simulink model "untitled"  (R2025b)
settings: Solver=VariableStepAuto  StartTime=0.0  StopTime=26  RelTol=1e-3
libraries: neural x35
(part 2 of 2)

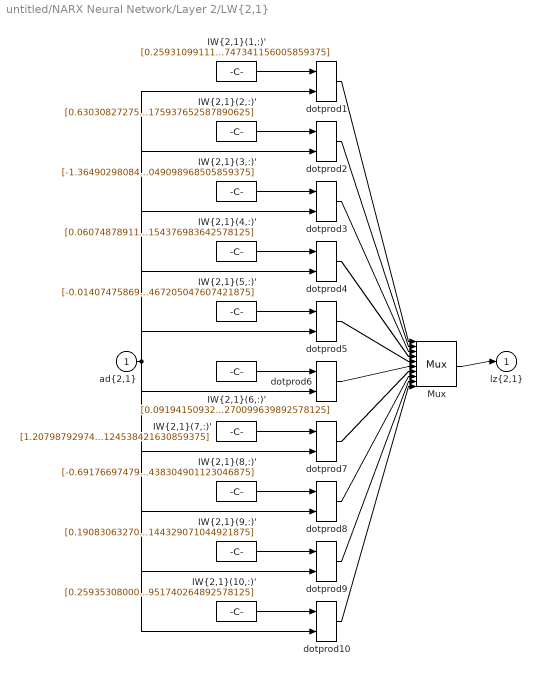
== system untitled/NARX Neural Network/Layer 2/LW{2,1} ==
  "ad{2,1}" : Inport  PortDimensions=10  SampleTime=1
      mask Display: e = 0.06;c1 = [120 230 180]/255;c2 = ([120 230 180]+0)/(256+128);c3 = ([120 230 180]+128)/(256+128);patch([0 1 1 0],[0 0 1 1],c1);patch([0 1 1 1-e 1-e 0+e],[0 0 1 1-e 0+e 0+e],c2);patch([0 0 1 1-e 0+e 0+e],[0 1 1 1-e 1-e 0+e],c3);plot([0 1 1 0 0],[0 0 1 1 0]);
  "IW{2,1}(1,:)'" : Constant  Value=[0.2593109911101532105703881825320422649383544921875;0.043027177460193015423595142010526615194976329803466796875;-0.031630578930780896274033153758864500559866428375244140625;-0.8946206870678163891597023393842391669750213623046875;-1.376635707680159637078531886800192296504974365234375;0.0101372112858142127134186694092932157218456268310546875;-0.036902676601514618204280537838712916709482669830322265625;0.07042545743955726245122406226073508150875568389892578125;0.126162243134557316981414487599977292120456695556640625;-0.6207380455155016019119784687063656747341156005859375]
      mask Display: e = 0.06;c1 = [120 150 230]/255;c2 = ([120 150 230]+0)/383;c3 = ([120 150 230]+128)/383;patch([0 1 1 0],[0 0 1 1],c1);patch([0 1 1 1-e 1-e 0+e],[0 0 1 1-e 0+e 0+e],c2);patch([0 0 1 1-e 0+e 0+e],[0 1 1 1-e 1-e 0+e],c3);plot([0 1 1 0 0],[0 0 1 1 0]);disp('weights');
  "IW{2,1}(10,:)'" : Constant  Value=[0.259353080009003644779141950493794865906238555908203125;0.0344788966224069126642604032895178534090518951416015625;-1.639734198097074990840837926953099668025970458984375;0.037171314064603451499113617728653480298817157745361328125;-0.044091665192930361294454399967435165308415889739990234375;0.113806681736434545104685867045191116631031036376953125;-0.0404618156560806740973390560611733235418796539306640625;0.0762493477749900117057535453568561933934688568115234375;-0.277877005672673871305988768654060550034046173095703125;0.047364494032463178019298766230349428951740264892578125]
      mask Display: e = 0.06;c1 = [120 150 230]/255;c2 = ([120 150 230]+0)/383;c3 = ([120 150 230]+128)/383;patch([0 1 1 0],[0 0 1 1],c1);patch([0 1 1 1-e 1-e 0+e],[0 0 1 1-e 0+e 0+e],c2);patch([0 0 1 1-e 0+e 0+e],[0 1 1 1-e 1-e 0+e],c3);plot([0 1 1 0 0],[0 0 1 1 0]);disp('weights');
  "IW{2,1}(2,:)'" : Constant  Value=[0.63030827275463219283579974216991104185581207275390625;0.95420909453976487935022987585398368537425994873046875;-0.0170684212993636071076242188837568392045795917510986328125;0.10423405085466287689488495971090742386877536773681640625;0.0933351443445988027125537200845428742468357086181640625;0.05706595557659464856836706303511164151132106781005859375;-0.0036970778483764979611969625494793945108540356159210205078125;0.0226284225386658120748872846661470248363912105560302734375;-0.169997488913500027774006184699828736484050750732421875;0.4467008606033611162189345122897066175937652587890625]
      mask Display: e = 0.06;c1 = [120 150 230]/255;c2 = ([120 150 230]+0)/383;c3 = ([120 150 230]+128)/383;patch([0 1 1 0],[0 0 1 1],c1);patch([0 1 1 1-e 1-e 0+e],[0 0 1 1-e 0+e 0+e],c2);patch([0 0 1 1-e 0+e 0+e],[0 1 1 1-e 1-e 0+e],c3);plot([0 1 1 0 0],[0 0 1 1 0]);disp('weights');
  "IW{2,1}(3,:)'" : Constant  Value=[-1.3649029808437316280134155022096820175647735595703125;-0.0099506250485993270882278949329702300019562244415283203125;0.004944580631372802632939045253124277223832905292510986328125;0.52636799453096261292017743471660651266574859619140625;0.0107608841966076625162873625640713726170361042022705078125;3.2396981083788300992409858736209571361541748046875;0.0175827063636769566346007565016407170332968235015869140625;-0.00844932741786058767730072105450744857080280780792236328125;-0.0488448562737805735967100417838082648813724517822265625;0.6284819327693680346413884763023816049098968505859375]
      mask Display: e = 0.06;c1 = [120 150 230]/255;c2 = ([120 150 230]+0)/383;c3 = ([120 150 230]+128)/383;patch([0 1 1 0],[0 0 1 1],c1);patch([0 1 1 1-e 1-e 0+e],[0 0 1 1-e 0+e 0+e],c2);patch([0 0 1 1-e 0+e 0+e],[0 1 1 1-e 1-e 0+e],c3);plot([0 1 1 0 0],[0 0 1 1 0]);disp('weights');
  "IW{2,1}(4,:)'" : Constant  Value=[0.060748789116446537394988780533822136931121349334716796875;-0.00794143061588940997463925697275044512934982776641845703125;-0.0246556586678514065569256530352504341863095760345458984375;-0.036168325016118781090046496728973579593002796173095703125;0.017769845931746054701338977110935957171022891998291015625;-0.00682202459217154215387335369769061799161136150360107421875;0.00478693571736033170183066687286554952152073383331298828125;1.828233176941406856741423325729556381702423095703125;-0.336457903351097209476705529596074484288692474365234375;-0.444354288008560083245157557030324824154376983642578125]
      mask Display: e = 0.06;c1 = [120 150 230]/255;c2 = ([120 150 230]+0)/383;c3 = ([120 150 230]+128)/383;patch([0 1 1 0],[0 0 1 1],c1);patch([0 1 1 1-e 1-e 0+e],[0 0 1 1-e 0+e 0+e],c2);patch([0 0 1 1-e 0+e 0+e],[0 1 1 1-e 1-e 0+e],c3);plot([0 1 1 0 0],[0 0 1 1 0]);disp('weights');
  "IW{2,1}(5,:)'" : Constant  Value=[-0.01407475869495870314518359833755312138237059116363525390625;-0.0813608715144924499185208333074115216732025146484375;0.1181201219432181648283375352548318915069103240966796875;0.76491096816797898849671355492318980395793914794921875;0.11204011842603171789090055199267226271331310272216796875;-0.385610136227055699809085353990667499601840972900390625;0.0940923757188020515318527259296388365328311920166015625;-0.152898200506478121329934083405532874166965484619140625;-0.0241401187729273873638913272543504717759788036346435546875;-1.02487649672637370912298138136975467205047607421875]
      mask Display: e = 0.06;c1 = [120 150 230]/255;c2 = ([120 150 230]+0)/383;c3 = ([120 150 230]+128)/383;patch([0 1 1 0],[0 0 1 1],c1);patch([0 1 1 1-e 1-e 0+e],[0 0 1 1-e 0+e 0+e],c2);patch([0 0 1 1-e 0+e 0+e],[0 1 1 1-e 1-e 0+e],c3);plot([0 1 1 0 0],[0 0 1 1 0]);disp('weights');
  "IW{2,1}(6,:)'" : Constant  Value=[0.09194150932908216888872487970729707740247249603271484375;0.00893170196256900909836939916885967249982059001922607421875;-0.00270216338763807316369902622454901575110852718353271484375;0.4384877115912220180149461157270707190036773681640625;-0.010539276489478908993557837447951897047460079193115234375;0.1074971903280156071414097596061765216290950775146484375;-0.0139268622037817708936291438703847234137356281280517578125;0.014467383049023820051903754801969625987112522125244140625;0.033730896861891353222251410670651239342987537384033203125;-0.47233994547981617007081922565703280270099639892578125]
      mask Display: e = 0.06;c1 = [120 150 230]/255;c2 = ([120 150 230]+0)/383;c3 = ([120 150 230]+128)/383;patch([0 1 1 0],[0 0 1 1],c1);patch([0 1 1 1-e 1-e 0+e],[0 0 1 1-e 0+e 0+e],c2);patch([0 0 1 1-e 0+e 0+e],[0 1 1 1-e 1-e 0+e],c3);plot([0 1 1 0 0],[0 0 1 1 0]);disp('weights');
  "IW{2,1}(7,:)'" : Constant  Value=[1.2079879297442683849794775596819818019866943359375;-0.96997720146081534142723512559314258396625518798828125;1.341993650625849188173788206768222153186798095703125;2.48313839798580904272284897160716354846954345703125;1.236241853293317038975374089204706251621246337890625;-2.98728747420875695439690389321185648441314697265625;0.99144276990696145190895549603737890720367431640625;-1.8470882435209095007166979485191404819488525390625;-0.39711441564978733342883288059965707361698150634765625;-1.9294405292739680302105398368439637124538421630859375]
      mask Display: e = 0.06;c1 = [120 150 230]/255;c2 = ([120 150 230]+0)/383;c3 = ([120 150 230]+128)/383;patch([0 1 1 0],[0 0 1 1],c1);patch([0 1 1 1-e 1-e 0+e],[0 0 1 1-e 0+e 0+e],c2);patch([0 0 1 1-e 0+e 0+e],[0 1 1 1-e 1-e 0+e],c3);plot([0 1 1 0 0],[0 0 1 1 0]);disp('weights');
  "IW{2,1}(8,:)'" : Constant  Value=[-0.6917669747991321838043177194776944816112518310546875;0.02005886442724380547275586650357581675052642822265625;0.2344520490258656664206426967211882583796977996826171875;0.16810169695141408130467652881634421646595001220703125;-0.0161572705531280273738570230079858447425067424774169921875;-0.1757694695147239138943717762231244705617427825927734375;-0.021758463862406492161927218376149539835751056671142578125;0.046202714262242240705891305196928442455828189849853515625;0.92224582634424034921494239824824035167694091796875;-0.57227723426191967615039857264491729438304901123046875]
      mask Display: e = 0.06;c1 = [120 150 230]/255;c2 = ([120 150 230]+0)/383;c3 = ([120 150 230]+128)/383;patch([0 1 1 0],[0 0 1 1],c1);patch([0 1 1 1-e 1-e 0+e],[0 0 1 1-e 0+e 0+e],c2);patch([0 0 1 1-e 0+e 0+e],[0 1 1 1-e 1-e 0+e],c3);plot([0 1 1 0 0],[0 0 1 1 0]);disp('weights');
  "IW{2,1}(9,:)'" : Constant  Value=[0.1908306327012936065568027288463781587779521942138671875;-0.0182508750380459862372450885459329583682119846343994140625;0.006372142546187395568957345659555357997305691242218017578125;-0.071890224988197803934752982968348078429698944091796875;0.044783945745097551716096262452992959879338741302490234375;0.026064510211621379209834259427225333638489246368408203125;-0.94180942639733522536715781825478188693523406982421875;-0.02284578978884177491437412754748947918415069580078125;-0.201690086770057452891791172078228555619716644287109375;0.63128763532050136131346107504214160144329071044921875]
      mask Display: e = 0.06;c1 = [120 150 230]/255;c2 = ([120 150 230]+0)/383;c3 = ([120 150 230]+128)/383;patch([0 1 1 0],[0 0 1 1],c1);patch([0 1 1 1-e 1-e 0+e],[0 0 1 1-e 0+e 0+e],c2);patch([0 0 1 1-e 0+e 0+e],[0 1 1 1-e 1-e 0+e],c3);plot([0 1 1 0 0],[0 0 1 1 0]);disp('weights');
  Mux : Mux  Inputs=10
      mask Display: e = 0.06;c1 = [120 150 230]/255;c2 = ([120 150 230]+0)/383;c3 = ([120 150 230]+128)/383;patch([0 1 1 0],[0 0 1 1],c1);patch([0 1 1 1-e 1-e 0+e],[0 0 1 1-e 0+e 0+e],c2);patch([0 0 1 1-e 0+e 0+e],[0 1 1 1-e 1-e 0+e],c3);plot([0 1 1 0 0],[0 0 1 1 0]);disp('Mux');
  dotprod{1..10} (10 alike) : neural/Weight Functions/dotprod
  "lz{2,1}" : Outport
      mask Display: e = 0.06;c1 = [120 230 180]/255;c2 = ([120 230 180]+0)/(256+128);c3 = ([120 230 180]+128)/(256+128);patch([0 1 1 0],[0 0 1 1],c1);patch([0 1 1 1-e 1-e 0+e],[0 0 1 1-e 0+e 0+e],c2);patch([0 0 1 1-e 0+e 0+e],[0 1 1 1-e 1-e 0+e],c3);plot([0 1 1 0 0],[0 0 1 1 0]);
  wires:
  "IW{2,1}(1,:)'"/1 -> dotprod1/1
  "ad{2,1}"/1 -> dotprod1/2, dotprod2/2, dotprod3/2, dotprod4/2, dotprod5/2, dotprod6/2, dotprod7/2, dotprod8/2, dotprod9/2, dotprod10/2
  dotprod1/1 -> Mux/1
  "IW{2,1}(2,:)'"/1 -> dotprod2/1
  dotprod2/1 -> Mux/2
  "IW{2,1}(3,:)'"/1 -> dotprod3/1
  dotprod3/1 -> Mux/3
  "IW{2,1}(4,:)'"/1 -> dotprod4/1
  dotprod4/1 -> Mux/4
  "IW{2,1}(5,:)'"/1 -> dotprod5/1
  dotprod5/1 -> Mux/5
  "IW{2,1}(6,:)'"/1 -> dotprod6/1
  dotprod6/1 -> Mux/6
  "IW{2,1}(7,:)'"/1 -> dotprod7/1
  dotprod7/1 -> Mux/7
  "IW{2,1}(8,:)'"/1 -> dotprod8/1
  dotprod8/1 -> Mux/8
  "IW{2,1}(9,:)'"/1 -> dotprod9/1
  dotprod9/1 -> Mux/9
  "IW{2,1}(10,:)'"/1 -> dotprod10/1
  dotprod10/1 -> Mux/10
  Mux/1 -> "lz{2,1}"/1
